simulink model "Mapping_cs"  (R2019a)
settings: Solver=ode5  StartTime=0.0  StopTime=inf  FixedStep=1/20  RelTol=1e-3
PreLoadFcn:
  | mbxruntime.callbacks.PreLoadFcn(bdroot);
PostLoadFcn:
  | mbxruntime.callbacks.PostLoadFcn(bdroot);
InitFcn:
  | mbxruntime.callbacks.InitFcn(bdroot);
StartFcn:
  | mbxruntime.callbacks.StartFcn(bdroot);
StopFcn:
  | mbxruntime.callbacks.StopFcn(bdroot);
model workspace: external: MAT-File .\Mapping_cs_hws.mat (data not in the file)
undefined symbols (not defined in the file or in its folder): InitImageOutputDir, Mapping_cs_BMW_X5_SUV_1_Path_pathUniqueID, Mapping_cs_BMW_X5_SUV_1_SpeedProfile_speedProfileUniqueID, mbxruntime
libraries: PreScanUsefulBlocks x1, adeye_lib x1
(part 2 of 2)

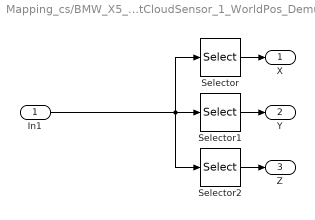
== system Mapping_cs/BMW_X5_SUV_1/PointCloudSensor_1_WorldPos_Demux ==
  In1 : Inport
  Selector : Selector  NumberOfDimensions=2  InputPortWidth=3  IndexOptions=Index vector (dialog),Index vector (dialog)  Indices=-1,offset+1:(offset+hres)  OutputSizes=1,1
  Selector1 : Selector  NumberOfDimensions=2  InputPortWidth=3  IndexOptions=Index vector (dialog),Index vector (dialog)  Indices=-1,(offset+hres+1):(offset+2*hres)  OutputSizes=1,1
  Selector2 : Selector  NumberOfDimensions=2  InputPortWidth=3  IndexOptions=Index vector (dialog),Index vector (dialog)  Indices=-1,(offset+2*hres+1):(offset+3*hres)  OutputSizes=1,1
  X : Outport
  Y : Outport  Port=2
  Z : Outport  Port=3
  wires:
  Selector2/1 -> Z/1
  Selector1/1 -> Y/1
  Selector/1 -> X/1
  In1/1 -> Selector2/1, Selector/1, Selector1/1

== system Mapping_cs/BMW_X5_SUV_1/PointCloudSensor_2_Intensity_Demux ==
  In1 : Inport
  Selector3 : Selector  NumberOfDimensions=2  InputPortWidth=3  IndexOptions=Index vector (dialog),Index vector (dialog)  Indices=-1,offset+1:(offset+hres)  OutputSizes=1,1
  Intensity : Outport
  wires:
  Selector3/1 -> Intensity/1
  In1/1 -> Selector3/1

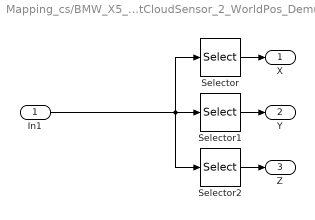
== system Mapping_cs/BMW_X5_SUV_1/PointCloudSensor_2_WorldPos_Demux ==
  In1 : Inport
  Selector : Selector  NumberOfDimensions=2  InputPortWidth=3  IndexOptions=Index vector (dialog),Index vector (dialog)  Indices=-1,offset+1:(offset+hres)  OutputSizes=1,1
  Selector1 : Selector  NumberOfDimensions=2  InputPortWidth=3  IndexOptions=Index vector (dialog),Index vector (dialog)  Indices=-1,(offset+hres+1):(offset+2*hres)  OutputSizes=1,1
  Selector2 : Selector  NumberOfDimensions=2  InputPortWidth=3  IndexOptions=Index vector (dialog),Index vector (dialog)  Indices=-1,(offset+2*hres+1):(offset+3*hres)  OutputSizes=1,1
  X : Outport
  Y : Outport  Port=2
  Z : Outport  Port=3
  wires:
  Selector2/1 -> Z/1
  Selector1/1 -> Y/1
  Selector/1 -> X/1
  In1/1 -> Selector2/1, Selector/1, Selector1/1

== system Mapping_cs/BMW_X5_SUV_1/PointCloudSensor_3_Intensity_Demux ==
  In1 : Inport
  Selector3 : Selector  NumberOfDimensions=2  InputPortWidth=3  IndexOptions=Index vector (dialog),Index vector (dialog)  Indices=-1,offset+1:(offset+hres)  OutputSizes=1,1
  Intensity : Outport
  wires:
  Selector3/1 -> Intensity/1
  In1/1 -> Selector3/1

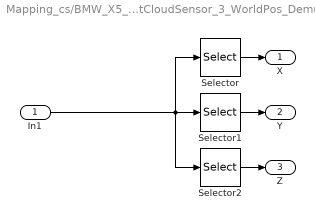
== system Mapping_cs/BMW_X5_SUV_1/PointCloudSensor_3_WorldPos_Demux ==
  In1 : Inport
  Selector : Selector  NumberOfDimensions=2  InputPortWidth=3  IndexOptions=Index vector (dialog),Index vector (dialog)  Indices=-1,offset+1:(offset+hres)  OutputSizes=1,1
  Selector1 : Selector  NumberOfDimensions=2  InputPortWidth=3  IndexOptions=Index vector (dialog),Index vector (dialog)  Indices=-1,(offset+hres+1):(offset+2*hres)  OutputSizes=1,1
  Selector2 : Selector  NumberOfDimensions=2  InputPortWidth=3  IndexOptions=Index vector (dialog),Index vector (dialog)  Indices=-1,(offset+2*hres+1):(offset+3*hres)  OutputSizes=1,1
  X : Outport
  Y : Outport  Port=2
  Z : Outport  Port=3
  wires:
  Selector2/1 -> Z/1
  Selector1/1 -> Y/1
  Selector/1 -> X/1
  In1/1 -> Selector2/1, Selector/1, Selector1/1

== system Mapping_cs/BMW_X5_SUV_1/PointCloudSensor_4_Intensity_Demux ==
  In1 : Inport
  Selector3 : Selector  NumberOfDimensions=2  InputPortWidth=3  IndexOptions=Index vector (dialog),Index vector (dialog)  Indices=-1,offset+1:(offset+hres)  OutputSizes=1,1
  Intensity : Outport
  wires:
  Selector3/1 -> Intensity/1
  In1/1 -> Selector3/1

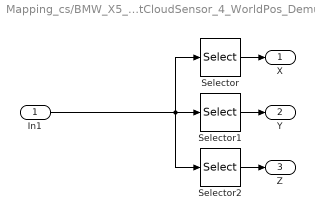
== system Mapping_cs/BMW_X5_SUV_1/PointCloudSensor_4_WorldPos_Demux ==
  In1 : Inport
  Selector : Selector  NumberOfDimensions=2  InputPortWidth=3  IndexOptions=Index vector (dialog),Index vector (dialog)  Indices=-1,offset+1:(offset+hres)  OutputSizes=1,1
  Selector1 : Selector  NumberOfDimensions=2  InputPortWidth=3  IndexOptions=Index vector (dialog),Index vector (dialog)  Indices=-1,(offset+hres+1):(offset+2*hres)  OutputSizes=1,1
  Selector2 : Selector  NumberOfDimensions=2  InputPortWidth=3  IndexOptions=Index vector (dialog),Index vector (dialog)  Indices=-1,(offset+2*hres+1):(offset+3*hres)  OutputSizes=1,1
  X : Outport
  Y : Outport  Port=2
  Z : Outport  Port=3
  wires:
  Selector2/1 -> Z/1
  Selector1/1 -> Y/1
  Selector/1 -> X/1
  In1/1 -> Selector2/1, Selector/1, Selector1/1

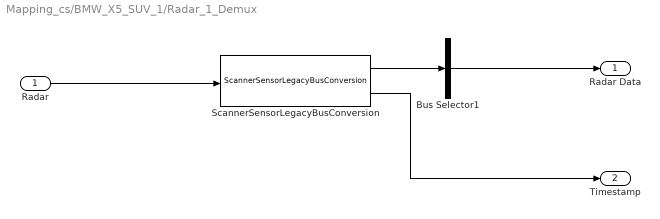
== system Mapping_cs/BMW_X5_SUV_1/Radar_1_Demux ==
  Radar : Inport
  Bus Selector1 : BusSelector  OutputSignals=ActiveBeamID[-],Range[m],DopplerVelocity[ms-1],DopplerVelocityX[ms-1],DopplerVelocityY[ms-1],DopplerVelocityZ[ms-1],Theta[deg],Phi[deg],TargetID[-],TargetTypeID[-],EnergyLoss[dB],Alpha[deg],Beta[deg]  OutputAsBus=on
  ScannerSensorLegacyBusConversion : PreScanUsefulBlocks/ScannerSensorLegacyBusConversion  MAXMESSAGES=MAXMESSAGES
  Radar Data : Outport
  Timestamp : Outport  Port=2
  wires:
  ScannerSensorLegacyBusConversion/2 -> Timestamp/1
  Bus Selector1/1 -> Radar Data/1
  ScannerSensorLegacyBusConversion/1 -> Bus Selector1/1
  Radar/1 -> ScannerSensorLegacyBusConversion/1

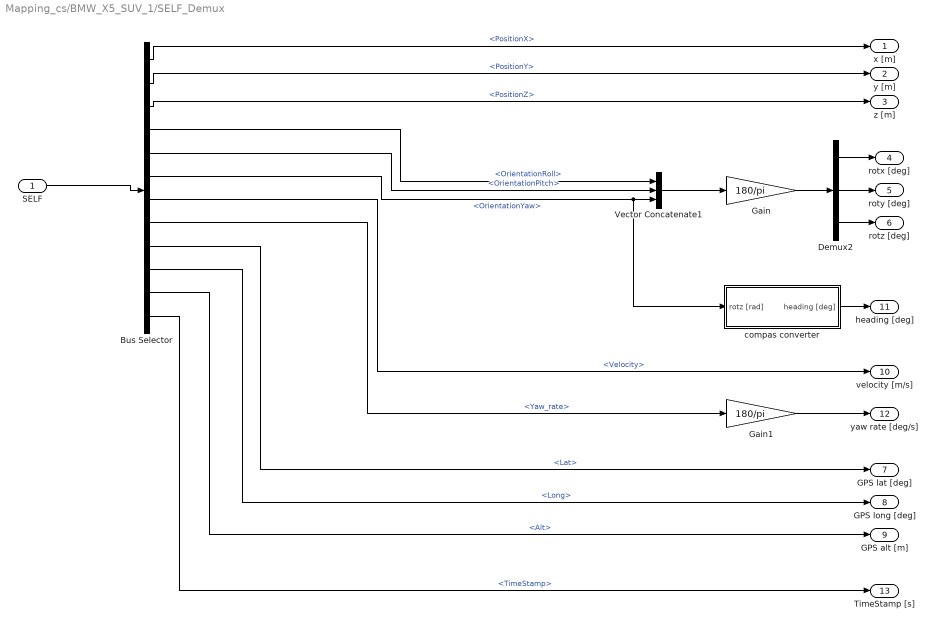
== system Mapping_cs/BMW_X5_SUV_1/SELF_Demux ==
  SELF : Inport  OutDataTypeStr=Bus: PRESCAN_SELFSENSORDATA
  Bus Selector : BusSelector  OutputSignals=PositionX,PositionY,PositionZ,OrientationRoll,OrientationPitch,OrientationYaw,Velocity,Yaw_rate,Lat,Long,Alt,TimeStamp
  Demux2 : Demux  Outputs=3
  Gain : Gain  Gain=180/pi
  Gain1 : Gain  Gain=180/pi
  Vector Concatenate1 : Concatenate  NumInputs=3
  compas converter : Subsystem
  x [m] : Outport
  y [m] : Outport  Port=2
  z [m] : Outport  Port=3
  rotx [deg] : Outport  Port=4
  roty [deg] : Outport  Port=5
  rotz [deg] : Outport  Port=6
  GPS lat [deg] : Outport  Port=7
  GPS long [deg] : Outport  Port=8
  GPS alt [m] : Outport  Port=9
  velocity [m/s] : Outport  Port=10
  heading [deg] : Outport  Port=11
  yaw rate [deg/s] : Outport  Port=12
  TimeStamp [s] : Outport  Port=13
  wires:
  Bus Selector/12 -> TimeStamp [s]/1  "<TimeStamp>"
  Bus Selector/11 -> GPS alt [m]/1  "<Alt>"
  Bus Selector/10 -> GPS long [deg]/1  "<Long>"
  Bus Selector/9 -> GPS lat [deg]/1  "<Lat>"
  Bus Selector/8 -> Gain1/1  "<Yaw_rate>"
  Bus Selector/7 -> velocity [m/s]/1  "<Velocity>"
  Bus Selector/6 -> compas converter/1(rotz [rad]), Vector Concatenate1/3  "<OrientationYaw>"
  Bus Selector/5 -> Vector Concatenate1/2  "<OrientationPitch>"
  Bus Selector/4 -> Vector Concatenate1/1  "<OrientationRoll>"
  Vector Concatenate1/1 -> Gain/1
  Bus Selector/3 -> z [m]/1  "<PositionZ>"
  Bus Selector/2 -> y [m]/1  "<PositionY>"
  Bus Selector/1 -> x [m]/1  "<PositionX>"
  SELF/1 -> Bus Selector/1
  Gain/1 -> Demux2/1
  Demux2/1 -> rotx [deg]/1
  Demux2/2 -> roty [deg]/1
  Demux2/3 -> rotz [deg]/1
  compas converter/1(heading [deg]) -> heading [deg]/1
  Gain1/1 -> yaw rate [deg/s]/1

== system Mapping_cs/BMW_X5_SUV_1/SELF_Demux/compas converter ==
  rotz [rad] : Inport
  cart2compas : Subsystem
  rad2deg : Gain  Gain=180/pi
  heading [deg] : Outport
  wires:
  rad2deg/1 -> cart2compas/1(Angle [deg])
  rotz [rad]/1 -> rad2deg/1
  cart2compas/1(heading [deg]) -> heading [deg]/1

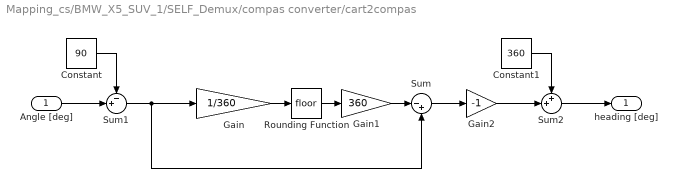
== system Mapping_cs/BMW_X5_SUV_1/SELF_Demux/compas converter/cart2compas ==
  Angle [deg] : Inport
  Constant : Constant  Value=90
  Constant1 : Constant  Value=360
  Gain : Gain  Gain=1/360
  Gain1 : Gain  Gain=360
  Gain2 : Gain  Gain=-1
  Rounding Function : Rounding
  Sum : Sum  Inputs=|-+
  Sum1 : Sum  Inputs=-+|
  Sum2 : Sum  Inputs=++|
  heading [deg] : Outport
  wires:
  Gain/1 -> Rounding Function/1
  Rounding Function/1 -> Gain1/1
  Gain1/1 -> Sum/1
  Angle [deg]/1 -> Sum1/2
  Sum/1 -> Gain2/1
  Sum1/1 -> Gain/1, Sum/2
  Constant/1 -> Sum1/1
  Gain2/1 -> Sum2/2
  Constant1/1 -> Sum2/1
  Sum2/1 -> heading [deg]/1
